simulink subsystem "encoder"  (R2022b)
settings: Solver=VariableStepAuto  StartTime=0.0  StopTime=10.0  RelTol=1e-3
libraries: arduinosensorlib x2
settings Model: Creator=miriamfreiriasanjuan  LastModifiedBy=miriamfreiriasanjuan

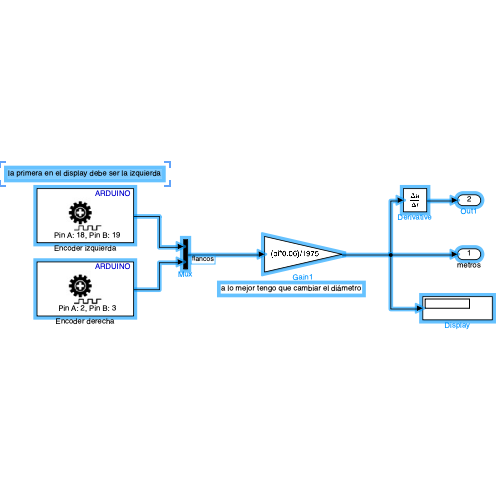
[thumbnail: Simulink's stored preview of the top-level diagram]
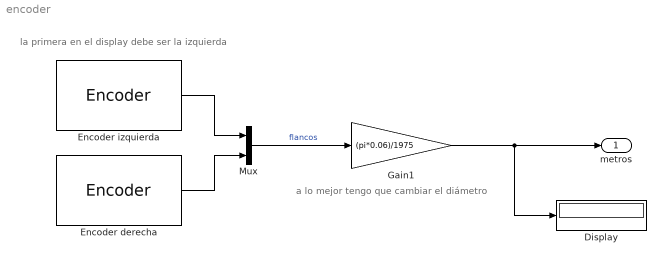
== system encoder ==
  note: a lo mejor tengo que cambiar el diámetro
  note: la primera en el display debe ser la izquierda
  Display : Display
  Encoder derecha : arduinosensorlib/Encoder  InputA=2  InputB=3  Mode=No reset  SampleTime=-1
  Encoder izquierda : arduinosensorlib/Encoder  InputA=18  InputB=19  Mode=No reset  SampleTime=-1
  Gain1 : Gain  Gain=(pi*0.06)/1975  ParamDataTypeStr=double  OutDataTypeStr=double
  Mux : Mux  Inputs=2
  metros : Outport
  wires:
  Encoder izquierda/1 -> Mux/1
  Gain1/1 -> metros/1, Display/1
  Encoder derecha/1 -> Mux/2
  Mux/1 -> Gain1/1  "flancos"
